simulink model "model_bins"  (R2014a)
settings: Solver=ode23s  StartTime=0.0  StopTime=1.0  MaxStep=0.001  RelTol=1e-3
settings Model: Creator=me  LastModifiedBy=me

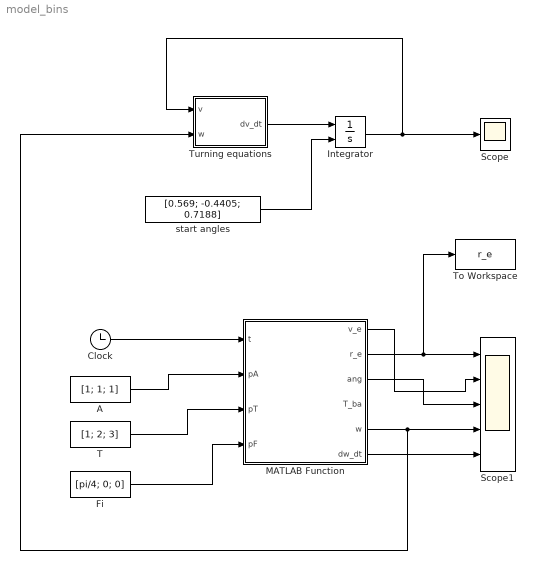
== system model_bins ==
  A : Constant  Value=[1; 1; 1]
  Clock : Clock
  Fi : Constant  Value=[pi/4; 0; 0]
  Integrator : Integrator  InitialConditionSource=external
  MATLAB Function : MATLAB Function  TreatAsAtomicUnit=on
  Scope : Scope
      settings: TimeRange=1  YMin=-4  YMax=3  MaxDataPoints=50000
  Scope1 : Scope  NumInputPorts=5
      settings: TimeRange=1  YMin=-1~-10~-2~-10~-1000  YMax=1~10~4~30~1000  MaxDataPoints=50000
  T : Constant  Value=[1; 2; 3]
  To Workspace : ToWorkspace  VariableName=r_e  SampleTime=-1
  Turning equations : MATLAB Function  TreatAsAtomicUnit=on
  start angles : Constant  Value=[0.569; -0.4405; 0.7188]
  wires:
  Turning equations/1(dv_dt) -> Integrator/1
  Integrator/1 -> Scope/1, Turning equations/1(v)
  start angles/1 -> Integrator/2
  A/1 -> MATLAB Function/2(pA)
  Clock/1 -> MATLAB Function/1(t)
  T/1 -> MATLAB Function/3(pT)
  Fi/1 -> MATLAB Function/4(pF)
  MATLAB Function/2(r_e) -> To Workspace/1, Scope1/1
  MATLAB Function/1(v_e) -> Scope1/2
  MATLAB Function/3(ang) -> Scope1/3
  MATLAB Function/5(w) -> Turning equations/2(w), Scope1/4
  MATLAB Function/6(dw_dt) -> Scope1/5

== matlab function model_bins/MATLAB Function ==
  data: v_e output; t input; r_e output; ang output; T_ba output; pA input; pT input; pF input; w output; dw_dt output
function [v_e, r_e, ang, T_ba, w, dw_dt] = fcn(t, pA, pT, pF)
%#codegen

    [r_e, v_e, w, dw_dt, T_ba, ang] = f_motion_model(t, pA, pT, pF);

end

== matlab function model_bins/Turning equations ==
  data: v input; w input; dv_dt output
function dv_dt = fcn(v, w)
%#codegen
dv_dt = f_turning_by_Euler(v, w);
end
